simulink model "L3_Sim_CSC_1"  (R2023b)
settings: Solver=VariableStepAuto  StartTime=0.0  StopTime=1  RelTol=1e-3
libraries: commcrc2 x2, commrandsrc3 x1, commchan3 x1, dspmathops x1, commsink2 x1
settings Model: Creator=Liu  LastModifiedBy=Liu

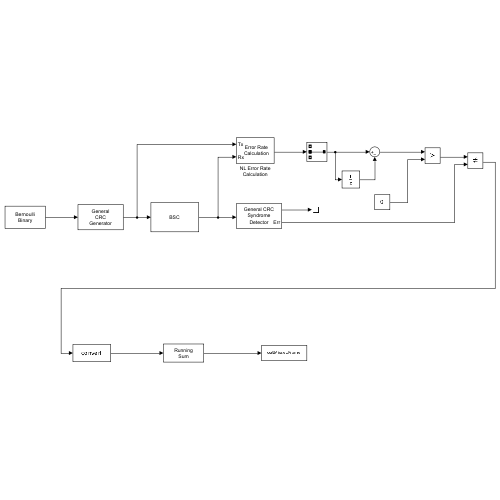
[thumbnail: Simulink's stored preview of the top-level diagram]
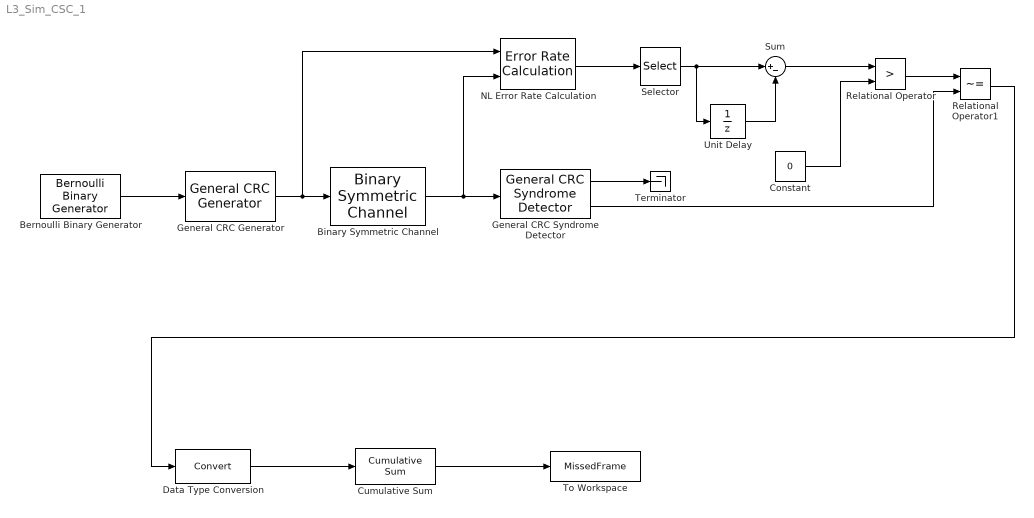
== system L3_Sim_CSC_1 ==
  Bernoulli Binary Generator : commrandsrc3/Bernoulli Binary Generator  ProbabilityOfZero=0.5  SeedSource=Parameter  Seed=61  SampleTime=1/1600000  SamplesPerFrame=16  OutputDataType=double  SimulateUsing=Interpreted execution
  Binary Symmetric Channel : commchan3/Binary Symmetric Channel  ErrorProbability=BER  ErrorVectorOutputPort=off  OutputDataType=double  OutputDataTypeSL=double  Seed=71  SimulateUsing=Code generation
  Constant : Constant  Value=0
  Cumulative Sum : dspmathops/Cumulative Sum  dim=Channels (running sum)  InputProcessing=Columns as channels (frame based)  reset_popup=None  roundingMode=Floor  overflowMode=off  outputDataTypeStr=Inherit: Same as accumulator  outputMin=[]  outputMax=[]  outputLastDataTypeStr=Inherit: Same as accumulator
  Data Type Conversion : DataTypeConversion  SaturateOnIntegerOverflow=off  RndMeth=Floor
  General CRC Generator : commcrc2/General CRC Generator  genPoly=[1 0 0 1 1 0 0 0 1]  iniStates=0  directMethod=off  reflectInputBytes=off  reflectChecksums=off  finalXOR=0  numChecksums=1
  General CRC Syndrome Detector : commcrc2/General CRC Syndrome Detector  genPoly=[1 0 0 1 1 0 0 0 1]  iniStates=0  directMethod=off  reflectInputBytes=off  reflectChecksums=off  finalXOR=0  numChecksums=1
  NL Error Rate Calculation : commsink2/Error Rate Calculation  N=0  st_delay=0  cp_mode=Entire frame  subframe=[]  PMode=Port  WsName=ErrorVec  RsMode2=off  stop=off  numErr=100  maxBits=1e6
  Relational Operator : RelationalOperator  Operator=>  OutDataTypeStr=boolean  RndMeth=Simplest  InputSameDT=off
  Relational Operator1 : RelationalOperator  Operator=~=  OutDataTypeStr=boolean  RndMeth=Simplest  InputSameDT=off
  Selector : Selector  InputPortWidth=3  IndexOptions=Index vector (dialog)  Indices=[2]  OutputSizes=1
  Sum : Sum  Inputs=|+-
  Terminator : Terminator
  To Workspace : ToWorkspace  VariableName=MissedFrame  SampleTime=-1
      settings: Save2DSignal=2-D array (concatenate along first dimension)
  Unit Delay : UnitDelay  SampleTime=-1  HasFrameUpgradeWarning=on
  wires:
  Bernoulli Binary Generator/1 -> General CRC Generator/1
  General CRC Generator/1 -> NL Error Rate Calculation/1, Binary Symmetric Channel/1
  Binary Symmetric Channel/1 -> NL Error Rate Calculation/2, General CRC Syndrome Detector/1
  NL Error Rate Calculation/1 -> Selector/1
  General CRC Syndrome Detector/1 -> Terminator/1
  Selector/1 -> Unit Delay/1, Sum/1
  Unit Delay/1 -> Sum/2
  Sum/1 -> Relational Operator/1
  Constant/1 -> Relational Operator/2
  Relational Operator/1 -> Relational Operator1/1
  General CRC Syndrome Detector/2 -> Relational Operator1/2
  Cumulative Sum/1 -> To Workspace/1
  Data Type Conversion/1 -> Cumulative Sum/1
  Relational Operator1/1 -> Data Type Conversion/1
